simulink model "ASM_Traffic_A11"  (R2026a)
settings: Solver=ode1  StartTime=SIM.tstart.v  StopTime=SIM.tend.v  FixedStep=SIM.StepSize.v
PostLoadFcn:
  | if any(exist('dsrtsu_mdlpostloadfcn', 'file') ~= 0), dsrtsu_mdlpostloadfcn('Execute', bdroot); end
  | try, asm_mdl_postloadfcn(bdroot, 'UpdateModel', 3600); catch, disp(lasterr); end,
InitFcn:
  | , if any(exist('rtifpga_mdlclblib', 'file') ~= 0), rtifpga_mdlclblib('Init', bdroot); end,
  | , if any(exist('dsmpb_private', 'file') ~= 0), dsmpb_private('dsmpb_mdlclblib', 'Init', bdroot); end,
undefined symbols (not defined in the file): _to_, a0b2, ASM_BrakeHydraulics_DemoSystems, ASM_VehicleDynamics_DemoSystems, b98103fe8ad365046cd0, BrakeCircuit, controllerConfig, CPT, Crankshaft, DiscIntNeverNeededParam, dsmsi, FinalDriveAssembly, instance, MDL, ModeSignals, mu, Pos_BrakePedal_Maneuver, rad, RefSignals, s_to_rpm, SIM, SoftECU, Suspension, Tire, Transmission
libraries: ASM_Traffic_lib x135, simulink x98, ASM_Utils_lib x77, ASM_VehicleDynamics_lib x70, ASM_Environment_lib x22, dsmpblib x20, dsmsilib x15, MDLD_Utils_lib x10, ASM_BrakeHydraulics_lib x3, sl_discontinuities x2
(part 63 of 63)

== system ASM_Traffic_A11/VehicleDynamics/Plant/VehicleDynamics/VehicleMovement/ASMSignalCollector/Vehicle_Movement_Info_Car/Accelerations/RelativeAcceleration ==
  q_Wheel_dt2[q1_Front;q2_Front;q1_Rear;q2_Rear][] : Inport
  ASMBUS_VehicleDynamics_Suspension : Inport  Port=2
  Displ_SteeringRod_dt2[m|s2] : Inport  Port=3
  Bus Selector1 : BusSelector  OutputSignals=SuspensionRear.SuspensionKinematicsRear.Kinematics_Left.Position_Left.Pos_Left_Wheel_dqL[x;y;z][],SuspensionRear.SuspensionKinematicsRear.Kinematics_Left.Position_Left.Pos_Left_Wheel_dqR[x;y;z][],SuspensionRear.SuspensionKinematicsRear.Kinematics_Left.Position_Left.Pos_Left_Wheel_dDispl_SteeringRod[x;y;z][],SuspensionRear.SuspensionKinematicsRear.Kinematics_Right.Position_Right.Pos_Right_Wheel_dqL[x;y;z][],SuspensionRear.SuspensionKinematicsRear.Kinematics_Right.Position_Right.Pos_Right_Wheel_dqR[x;y;z][],SuspensionRear.SuspensionKinematicsRear.Kinematics_Right.Position_Right.Pos_Right_Wheel_dDispl_SteeringRod[x;y;z][]
  Bus Selector2 : BusSelector  OutputSignals=SuspensionFront.SuspensionKinematicsFront.Kinematics_Left.Position_Left.Pos_Left_Wheel_dqL[x;y;z][],SuspensionFront.SuspensionKinematicsFront.Kinematics_Left.Position_Left.Pos_Left_Wheel_dqR[x;y;z][],SuspensionFront.SuspensionKinematicsFront.Kinematics_Left.Position_Left.Pos_Left_Wheel_dDispl_SteeringRod[x;y;z][],SuspensionFront.SuspensionKinematicsFront.Kinematics_Right.Position_Right.Pos_Right_Wheel_dqL[x;y;z][],SuspensionFront.SuspensionKinematicsFront.Kinematics_Right.Position_Right.Pos_Right_Wheel_dqR[x;y;z][],SuspensionFront.SuspensionKinematicsFront.Kinematics_Right.Position_Right.Pos_Right_Wheel_dDispl_SteeringRod[x;y;z][]
  Demux : Demux  Outputs=[1 1 1 1]
  Ground : Constant  Value=0
  RelativeAcceleration_FL : Subsystem
  RelativeAcceleration_FR : Subsystem
  RelativeAcceleration_RL : Subsystem
  RelativeAcceleration_RR : Subsystem
  Pos_FL_dt2[x;y;z][m|s2] : Outport  VectorParamsAs1DForOutWhenUnconnected=off
  Pos_FR_dt2[x;y;z][m|s2] : Outport  Port=2  VectorParamsAs1DForOutWhenUnconnected=off
  Pos_RL_dt2[x;y;z][m|s2] : Outport  Port=3  VectorParamsAs1DForOutWhenUnconnected=off
  Pos_RR_dt2[x;y;z][m|s2] : Outport  Port=4  VectorParamsAs1DForOutWhenUnconnected=off
  wires:
  Bus Selector1/6 -> RelativeAcceleration_RR/6(Pos_i_dqSteering[x;y;z][])  "<Pos_Right_Wheel_dDispl_SteeringRod[x;y;z][]>"
  Bus Selector1/5 -> RelativeAcceleration_RR/4(Pos_i_dq2[x;y;z][])  "<Pos_Right_Wheel_dqR[x;y;z][]>"
  Bus Selector1/4 -> RelativeAcceleration_RR/2(Pos_i_dq1[x;y;z][])  "<Pos_Right_Wheel_dqL[x;y;z][]>"
  Ground/1 -> RelativeAcceleration_RR/5(qSteering_dt2[m|s2]), RelativeAcceleration_RL/5(qSteering_dt2[m|s2])
  Bus Selector1/3 -> RelativeAcceleration_RL/6(Pos_i_dqSteering[x;y;z][])  "<Pos_Left_Wheel_dDispl_SteeringRod[x;y;z][]>"
  Bus Selector1/2 -> RelativeAcceleration_RL/4(Pos_i_dq2[x;y;z][])  "<Pos_Left_Wheel_dqR[x;y;z][]>"
  Bus Selector1/1 -> RelativeAcceleration_RL/2(Pos_i_dq1[x;y;z][])  "<Pos_Left_Wheel_dqL[x;y;z][]>"
  Bus Selector2/3 -> RelativeAcceleration_FL/6(Pos_i_dqSteering[x;y;z][])  "<Pos_Left_Wheel_dDispl_SteeringRod[x;y;z][]>"
  Demux/1 -> RelativeAcceleration_FL/1(q1_dt2[m|s2]), RelativeAcceleration_FR/1(q1_dt2[m|s2])
  Bus Selector2/6 -> RelativeAcceleration_FR/6(Pos_i_dqSteering[x;y;z][])  "<Pos_Right_Wheel_dDispl_SteeringRod[x;y;z][]>"
  Displ_SteeringRod_dt2[m|s2]/1 -> RelativeAcceleration_FL/5(qSteering_dt2[m|s2]), RelativeAcceleration_FR/5(qSteering_dt2[m|s2])
  Bus Selector2/5 -> RelativeAcceleration_FR/4(Pos_i_dq2[x;y;z][])  "<Pos_Right_Wheel_dqR[x;y;z][]>"
  Bus Selector2/4 -> RelativeAcceleration_FR/2(Pos_i_dq1[x;y;z][])  "<Pos_Right_Wheel_dqL[x;y;z][]>"
  Bus Selector2/2 -> RelativeAcceleration_FL/4(Pos_i_dq2[x;y;z][])  "<Pos_Left_Wheel_dqR[x;y;z][]>"
  Bus Selector2/1 -> RelativeAcceleration_FL/2(Pos_i_dq1[x;y;z][])  "<Pos_Left_Wheel_dqL[x;y;z][]>"
  ASMBUS_VehicleDynamics_Suspension/1 -> Bus Selector1/1, Bus Selector2/1
  RelativeAcceleration_FL/1(Pos_i_dt2[x;y;z][m|s2]) -> Pos_FL_dt2[x;y;z][m|s2]/1
  RelativeAcceleration_FR/1(Pos_i_dt2[x;y;z][m|s2]) -> Pos_FR_dt2[x;y;z][m|s2]/1
  RelativeAcceleration_RL/1(Pos_i_dt2[x;y;z][m|s2]) -> Pos_RL_dt2[x;y;z][m|s2]/1
  RelativeAcceleration_RR/1(Pos_i_dt2[x;y;z][m|s2]) -> Pos_RR_dt2[x;y;z][m|s2]/1
  Demux/2 -> RelativeAcceleration_FL/3(q2_dt2[m|s2]), RelativeAcceleration_FR/3(q2_dt2[m|s2])
  q_Wheel_dt2[q1_Front;q2_Front;q1_Rear;q2_Rear][]/1 -> Demux/1
  Demux/3 -> RelativeAcceleration_RR/1(q1_dt2[m|s2]), RelativeAcceleration_RL/1(q1_dt2[m|s2])
  Demux/4 -> RelativeAcceleration_RR/3(q2_dt2[m|s2]), RelativeAcceleration_RL/3(q2_dt2[m|s2])

== system ASM_Traffic_A11/VehicleDynamics/Plant/VehicleDynamics/VehicleMovement/ASMSignalCollector/Vehicle_Movement_Info_Car/Positions/VectorLabel ==
  in : Inport
  BusCreator : BusCreator  Inputs=3
  Demux : Demux  Outputs=3
      settings: DisplayOption=none
  out : Outport  VectorParamsAs1DForOutWhenUnconnected=off
  wires:
  in/1 -> Demux/1
  Demux/1 -> BusCreator/1  "Pos_x_Vehicle_CoorSys_E[m]"
  Demux/2 -> BusCreator/2  "Pos_y_Vehicle_CoorSys_E[m]"
  Demux/3 -> BusCreator/3  "Pos_z_Vehicle_CoorSys_E[m]"
  BusCreator/1 -> out/1  "Pos_Vehicle_CoorSys_E[x;y;z][m]"

== system ASM_Traffic_A11/VehicleDynamics/Plant/VehicleDynamics/VehicleMovement/ASMSignalCollector/Vehicle_Movement_Info_Car/Positions/VectorLabel2 ==
  in : Inport
  BusCreator : BusCreator  Inputs=3
  Demux : Demux  Outputs=3
      settings: DisplayOption=none
  out : Outport  VectorParamsAs1DForOutWhenUnconnected=off
  wires:
  BusCreator/1 -> out/1  "Angle_Vehicle_CoorSys_E[x;y;z][deg]"
  Demux/3 -> BusCreator/3  "Angle_Yaw_Vehicle_CoorSys_E[deg]"
  Demux/2 -> BusCreator/2  "Angle_Pitch_Vehicle_CoorSys_E[deg]"
  Demux/1 -> BusCreator/1  "Angle_Roll_Vehicle_CoorSys_E[deg]"
  in/1 -> Demux/1

== system ASM_Traffic_A11/VehicleDynamics/Plant/VehicleDynamics/VehicleMovement/ASMSignalCollector/Vehicle_Movement_Info_Car/Velocities/VectorLabel ==
  in : Inport
  BusCreator : BusCreator  Inputs=3
  Demux : Demux  Outputs=3
      settings: DisplayOption=none
  out : Outport  VectorParamsAs1DForOutWhenUnconnected=off
  wires:
  in/1 -> Demux/1
  Demux/1 -> BusCreator/1  "v_x_Vehicle_CoG[km|h]"
  Demux/2 -> BusCreator/2  "v_y_Vehicle_CoG[km|h]"
  Demux/3 -> BusCreator/3  "v_z_Vehicle_CoG[km|h]"
  BusCreator/1 -> out/1  "v_Vehicle_CoG[x;y;z][km|h]"

== system ASM_Traffic_A11/VehicleDynamics/Plant/VehicleDynamics/VehicleMovement/ASMSignalCollector/Vehicle_Movement_Info_Car/Velocities/VectorLabel3 ==
  in : Inport
  BusCreator : BusCreator  Inputs=3
  Demux : Demux  Outputs=3
      settings: DisplayOption=none
  out : Outport  VectorParamsAs1DForOutWhenUnconnected=off
  wires:
  BusCreator/1 -> out/1  "w_Vehicle_CoG[x;y;z][deg|s]"
  Demux/3 -> BusCreator/3  "YawRate_Vehicle_CoG[deg|s]"
  Demux/2 -> BusCreator/2  "PitchRate_Vehicle_CoG[deg|s]"
  Demux/1 -> BusCreator/1  "RollRate_Vehicle_CoG[deg|s]"
  in/1 -> Demux/1

== system ASM_Traffic_A11/VehicleDynamics/Plant/VehicleDynamics/VehicleMovement/ASMSignalCollector/Vehicle_Movement_Info_Car/Velocities/VectorLabel4 ==
  in : Inport
  BusCreator : BusCreator  Inputs=4
  Demux : Demux
      settings: DisplayOption=none
  out : Outport  VectorParamsAs1DForOutWhenUnconnected=off
  wires:
  Demux/4 -> BusCreator/4  "z_RR_Wheel_dt[m|s]"
  Demux/3 -> BusCreator/3  "z_RL_Wheel_dt[m|s]"
  Demux/2 -> BusCreator/2  "z_FR_Wheel_dt[m|s]"
  Demux/1 -> BusCreator/1  "z_FL_Wheel_dt[m|s]"
  BusCreator/1 -> out/1  "z_Wheel_dt[FL;FR;RL;RR][m|s]"
  in/1 -> Demux/1

== system ASM_Traffic_A11/VehicleDynamics/Plant/VehicleDynamics/VehicleMovement/ASMSignalCollector/Vehicle_Movement_Info_Car/Velocities/v_Vehicle_and_AngleSideSlip ==
  v_Vehicle[x;y][km|h] : Inport
  Demux : Demux  Outputs=[1 1]
  Math Function : Math  Operator=sqrt  SignedPower=on
  Math Function1 : Math  Operator=square  SignedPower=on
  NotZero : simulink/Logic and Bit Operations/Compare To Constant  relop=>  const=0.15  OutDataTypeStr=uint8
  Sum of Elements : Sum  Inputs=+
  Switch : Switch  Threshold=1  SaturateOnIntegerOverflow=off  InputSameDT=off
  Trigonometric Function : Trigonometry  Operator=atan2
  Zero : Constant  Value=0
  "[rad]_to_[deg]" : Gain  Gain=180/pi
  v_Vehicle[km|h] : Outport  VectorParamsAs1DForOutWhenUnconnected=off
  Angle_SideSlip_Vehicle[deg] : Outport  Port=2  VectorParamsAs1DForOutWhenUnconnected=off
  wires:
  Zero/1 -> Switch/3
  NotZero/1 -> Switch/2
  Switch/1 -> Angle_SideSlip_Vehicle[deg]/1
  Math Function/1 -> NotZero/1, v_Vehicle[km|h]/1
  Math Function1/1 -> Sum of Elements/1
  Sum of Elements/1 -> Math Function/1
  v_Vehicle[x;y][km|h]/1 -> Math Function1/1, Demux/1
  Trigonometric Function/1 -> "[rad]_to_[deg]"/1
  Demux/2 -> Trigonometric Function/1
  Demux/1 -> Trigonometric Function/2
  "[rad]_to_[deg]"/1 -> Switch/1

== system ASM_Traffic_A11/VehicleDynamics/Plant/VehicleDynamics/VehicleMovement/ASMSignalCollector/Vehicle_Movement_Info_Car/Accelerations/RelativeAcceleration/RelativeAcceleration_FL ==
  q1_dt2[m|s2] : Inport
  Pos_i_dq1[x;y;z][] : Inport  Port=2
  q2_dt2[m|s2] : Inport  Port=3
  Pos_i_dq2[x;y;z][] : Inport  Port=4
  qSteering_dt2[m|s2] : Inport  Port=5
  Pos_i_dqSteering[x;y;z][] : Inport  Port=6
  Product : Product  SaturateOnIntegerOverflow=on  OutDataTypeStr=Inherit: Same as first input
  Product1 : Product  SaturateOnIntegerOverflow=on  OutDataTypeStr=Inherit: Same as first input
  Product2 : Product  SaturateOnIntegerOverflow=on  OutDataTypeStr=Inherit: Same as first input
  Sum4 : Sum  Inputs=+++  SaturateOnIntegerOverflow=on
  Pos_i_dt2[x;y;z][m|s2] : Outport  VectorParamsAs1DForOutWhenUnconnected=off
  wires:
  Sum4/1 -> Pos_i_dt2[x;y;z][m|s2]/1
  q1_dt2[m|s2]/1 -> Product/1
  Pos_i_dq1[x;y;z][]/1 -> Product/2
  q2_dt2[m|s2]/1 -> Product1/1
  Pos_i_dq2[x;y;z][]/1 -> Product1/2
  Product/1 -> Sum4/1
  Product1/1 -> Sum4/2
  qSteering_dt2[m|s2]/1 -> Product2/1
  Pos_i_dqSteering[x;y;z][]/1 -> Product2/2
  Product2/1 -> Sum4/3

== system ASM_Traffic_A11/VehicleDynamics/Plant/VehicleDynamics/VehicleMovement/ASMSignalCollector/Vehicle_Movement_Info_Car/Accelerations/RelativeAcceleration/RelativeAcceleration_FR ==
  q1_dt2[m|s2] : Inport
  Pos_i_dq1[x;y;z][] : Inport  Port=2
  q2_dt2[m|s2] : Inport  Port=3
  Pos_i_dq2[x;y;z][] : Inport  Port=4
  qSteering_dt2[m|s2] : Inport  Port=5
  Pos_i_dqSteering[x;y;z][] : Inport  Port=6
  Product : Product  SaturateOnIntegerOverflow=on  OutDataTypeStr=Inherit: Same as first input
  Product1 : Product  SaturateOnIntegerOverflow=on  OutDataTypeStr=Inherit: Same as first input
  Product2 : Product  SaturateOnIntegerOverflow=on  OutDataTypeStr=Inherit: Same as first input
  Sum4 : Sum  Inputs=+++  SaturateOnIntegerOverflow=on
  Pos_i_dt2[x;y;z][m|s2] : Outport  VectorParamsAs1DForOutWhenUnconnected=off
  wires:
  Product2/1 -> Sum4/3
  Pos_i_dqSteering[x;y;z][]/1 -> Product2/2
  qSteering_dt2[m|s2]/1 -> Product2/1
  Product1/1 -> Sum4/2
  Product/1 -> Sum4/1
  Pos_i_dq2[x;y;z][]/1 -> Product1/2
  q2_dt2[m|s2]/1 -> Product1/1
  Pos_i_dq1[x;y;z][]/1 -> Product/2
  q1_dt2[m|s2]/1 -> Product/1
  Sum4/1 -> Pos_i_dt2[x;y;z][m|s2]/1

== system ASM_Traffic_A11/VehicleDynamics/Plant/VehicleDynamics/VehicleMovement/ASMSignalCollector/Vehicle_Movement_Info_Car/Accelerations/RelativeAcceleration/RelativeAcceleration_RL ==
  q1_dt2[m|s2] : Inport
  Pos_i_dq1[x;y;z][] : Inport  Port=2
  q2_dt2[m|s2] : Inport  Port=3
  Pos_i_dq2[x;y;z][] : Inport  Port=4
  qSteering_dt2[m|s2] : Inport  Port=5
  Pos_i_dqSteering[x;y;z][] : Inport  Port=6
  Product : Product  SaturateOnIntegerOverflow=on  OutDataTypeStr=Inherit: Same as first input
  Product1 : Product  SaturateOnIntegerOverflow=on  OutDataTypeStr=Inherit: Same as first input
  Product2 : Product  SaturateOnIntegerOverflow=on  OutDataTypeStr=Inherit: Same as first input
  Sum4 : Sum  Inputs=+++  SaturateOnIntegerOverflow=on
  Pos_i_dt2[x;y;z][m|s2] : Outport  VectorParamsAs1DForOutWhenUnconnected=off
  wires:
  Product2/1 -> Sum4/3
  Pos_i_dqSteering[x;y;z][]/1 -> Product2/2
  qSteering_dt2[m|s2]/1 -> Product2/1
  Product1/1 -> Sum4/2
  Product/1 -> Sum4/1
  Pos_i_dq2[x;y;z][]/1 -> Product1/2
  q2_dt2[m|s2]/1 -> Product1/1
  Pos_i_dq1[x;y;z][]/1 -> Product/2
  q1_dt2[m|s2]/1 -> Product/1
  Sum4/1 -> Pos_i_dt2[x;y;z][m|s2]/1

== system ASM_Traffic_A11/VehicleDynamics/Plant/VehicleDynamics/VehicleMovement/ASMSignalCollector/Vehicle_Movement_Info_Car/Accelerations/RelativeAcceleration/RelativeAcceleration_RR ==
  q1_dt2[m|s2] : Inport
  Pos_i_dq1[x;y;z][] : Inport  Port=2
  q2_dt2[m|s2] : Inport  Port=3
  Pos_i_dq2[x;y;z][] : Inport  Port=4
  qSteering_dt2[m|s2] : Inport  Port=5
  Pos_i_dqSteering[x;y;z][] : Inport  Port=6
  Product : Product  SaturateOnIntegerOverflow=on  OutDataTypeStr=Inherit: Same as first input
  Product1 : Product  SaturateOnIntegerOverflow=on  OutDataTypeStr=Inherit: Same as first input
  Product2 : Product  SaturateOnIntegerOverflow=on  OutDataTypeStr=Inherit: Same as first input
  Sum4 : Sum  Inputs=+++  SaturateOnIntegerOverflow=on
  Pos_i_dt2[x;y;z][m|s2] : Outport  VectorParamsAs1DForOutWhenUnconnected=off
  wires:
  Sum4/1 -> Pos_i_dt2[x;y;z][m|s2]/1
  q1_dt2[m|s2]/1 -> Product/1
  Pos_i_dq1[x;y;z][]/1 -> Product/2
  q2_dt2[m|s2]/1 -> Product1/1
  Pos_i_dq2[x;y;z][]/1 -> Product1/2
  Product/1 -> Sum4/1
  Product1/1 -> Sum4/2
  qSteering_dt2[m|s2]/1 -> Product2/1
  Pos_i_dqSteering[x;y;z][]/1 -> Product2/2
  Product2/1 -> Sum4/3

== matlab function ASM_Traffic_A11/AnimationInterface/ANIMATION_INTERFACE/Bounding_Boxes/EnableBoxVisualization/Move_Unused_Bounding_Boxes ==
  data: pos_x_out output; pos_y_out output; pos_z_out output; angle_x_out output; angle_y_out output; angle_z_out output; length_out output; width_out output; height_out output; pos_x_in input; pos_y_in input; pos_z_in input; angle_x_in input; angle_y_in input; angle_z_in input; length_in input; width_in input; height_in input
function [pos_x_out, pos_y_out, pos_z_out, angle_x_out, angle_y_out, angle_z_out, length_out, width_out, height_out] = ...
    Move_Unused_Bounding_Boxes(pos_x_in, pos_y_in, pos_z_in, angle_x_in, angle_y_in, angle_z_in, length_in, width_in, height_in)

pos_x_out   = pos_x_in;
pos_y_out   = pos_y_in;
pos_z_out   = pos_z_in;

angle_x_out = angle_x_in;
angle_y_out = angle_y_in;
angle_z_out = angle_z_in;

length_out  = length_in;
width_out   = width_in;
height_out  = height_in;

num_objects = length(pos_x_in);

for i = 1:num_objects
    if length_in(i) == 0.0
        % Move bounding box to [x, y, z] = [-1e9, -1e9, -1e9] since object
        % is not available
        pos_x_out(i) = -1e9;
        pos_y_out(i) = -1e9;
        pos_z_out(i) = -1e9;

        % Scale down bounding box
        length_out(i) = 0.1;
        width_out(i)  = 0.1;
        height_out(i) = 0.1;
    end
end

== matlab function ASM_Traffic_A11/Environment/Traffic/PlantModel/FellowMovement/ObjectParameters_Modified/MATLAB Function ==
  data: s_fellow_m input size=MDL.Traffic.MaxNumFellows.v; hitch_dist output size=MDL.Traffic.MaxNumFellows.v
function hitch_dist = calc_hitch_dist(s_fellow_m)
nFellows = numel(s_fellow_m);
hitch_dist = zeros(nFellows, 1);

for kk = 1:nFellows-1
    hitch_dist(kk) = abs(s_fellow_m(kk) - s_fellow_m(kk+1));
end %for kk
hitch_dist(nFellows) = 3.75;
end %calc_hitch_dist

== matlab function ASM_Traffic_A11/controller_subsys/assemble_problem ==
  data: t input; x input size=[5 1]; solverInputs output Bus: SolverInputBus; P input size=[19 41]; Xguess input size=[5 41]; Uguess input size=[3 40]; controllerConfig parameter; mu parameter
function solverInputs = assembleProblem( ...
    t, x, P, Xguess, Uguess, controllerConfig, mu)

warmStart.x = Xguess;
warmStart.u = Uguess;

ports = ecu.control.format_simulink_inputs( ...
    x, P, mu, warmStart, controllerConfig);

% Arrange fields in the solver adapter's input order.
solverInputs.lbx_0 = ports.lbx_0;
solverInputs.ubx_0 = ports.ubx_0;
solverInputs.parameter_traj = ports.parameter_traj;

solverInputs.lh = ports.lh;
solverInputs.uh = ports.uh;
solverInputs.lh_0 = ports.lh_0;
solverInputs.uh_0 = ports.uh_0;

solverInputs.x_init = ports.x_init;
solverInputs.u_init = ports.u_init;
solverInputs.iter_cap = double(controllerConfig.max_iter);

end

== matlab function ASM_Traffic_A11/controller_subsys/horizon_prep ==
  data: t input double size=1; P output; s input size=1; vx input size=1; Xguess input size=[205 1]; controllerConfig parameter; instance parameter
function P = buildHorizon( ...
    t, s, vx, Xguess, controllerConfig, instance)
% Build the stage parameters for the current controller execution.
assert(numel(Xguess) == 205);
Xmatrix = reshape(Xguess, 5, 41);
previousSpeedErrors = Xmatrix(3, 1:40);
% Use the existing A6 analytical reference and obstacle prediction.
P = ecu.scenario.prepare_horizon( ...
    instance, ...
    t, ...
    s, ...
    vx, ...
    previousSpeedErrors, ...
    controllerConfig);

end

== matlab function ASM_Traffic_A11/controller_subsys/warm_start/MATLAB Function ==
  data: X input; nextX output; U input; nextU output
function [nextX, nextU] = shiftWarmStart(X, U)
% Shift the previous solution using the shared MATLAB implementation.

warmStart = ecu.control.shift_warm_start(X, U);

nextX = warmStart.x;
nextU = warmStart.u;

end
